simulink model "s_c107m32k_vlbi"  (R2018a)
settings: Solver=VariableStepDiscrete  StartTime=0.0  StopTime=(2^15)*10  RelTol=1e-3
undefined symbols (not defined in the file): fft_stages, n_bits_xengs
libraries: xbsIndex_r4 x23049, casper_library_misc x45, xps_library x4, casper_library_scopes x3, simulink x2
(part 45 of 201)

== system s_c107m32k_vlbi/calc_ddc_pwr1/negedge ==
  In : Inport
  Convert : xbsIndex_r4/Convert  gui_display_data_type=Fixed-point  arith_type=Boolean  n_bits=8  bin_pt=6  float_type=Single  exp_bits=8  fraction_bits=24  quantization=Truncate  overflow=Wrap  en=off  latency=0  pipeline=off  dbl_ovrd=off  block_type=convert
      settings: xl_area=[0, 0, 0, 0, 0, 0, 0]  block_version=10.1.3
  Delay : xbsIndex_r4/Delay  rst=off  infoeditControl=Selection of Reset will increase slice count due to use of real FFs and instead of SRLs  en=off  latency=1  reg_retiming=off  dbl_ovrd=off  block_type=delay
      settings: xl_area=[0, 0, 0, 0, 0, 0, 0]
  Inverter1 : xbsIndex_r4/Inverter  en=off  latency=0  dbl_ovrd=off  block_type=inv
      settings: xl_area=[0, 0, 0, 0, 0, 0, 0]
  Logical : xbsIndex_r4/Logical  logical_function=AND  inputs=2  en=off  latency=0  precision=Full  arith_type=Unsigned  n_bits=8  bin_pt=2  align_bp=on  dbl_ovrd=off  block_type=logical
      settings: xl_area=[0, 0, 0, 0, 0, 0, 0]
  Out1 : Outport
  wires:
  Inverter1/1 -> Logical/2
  Logical/1 -> Convert/1
  In/1 -> Inverter1/1, Delay/1
  Delay/1 -> Logical/1
  Convert/1 -> Out1/1

== system s_c107m32k_vlbi/calc_fft_pwr0/negedge ==
  In : Inport
  Convert : xbsIndex_r4/Convert  gui_display_data_type=Fixed-point  arith_type=Boolean  n_bits=8  bin_pt=6  float_type=Single  exp_bits=8  fraction_bits=24  quantization=Truncate  overflow=Wrap  en=off  latency=0  pipeline=off  dbl_ovrd=off  block_type=convert
      settings: xl_area=[0, 0, 0, 0, 0, 0, 0]  block_version=10.1.3
  Delay : xbsIndex_r4/Delay  rst=off  infoeditControl=Selection of Reset will increase slice count due to use of real FFs and instead of SRLs  en=off  latency=1  reg_retiming=off  dbl_ovrd=off  block_type=delay
      settings: xl_area=[0, 0, 0, 0, 0, 0, 0]
  Inverter1 : xbsIndex_r4/Inverter  en=off  latency=0  dbl_ovrd=off  block_type=inv
      settings: xl_area=[0, 0, 0, 0, 0, 0, 0]
  Logical : xbsIndex_r4/Logical  logical_function=AND  inputs=2  en=off  latency=0  precision=Full  arith_type=Unsigned  n_bits=8  bin_pt=2  align_bp=on  dbl_ovrd=off  block_type=logical
      settings: xl_area=[0, 0, 0, 0, 0, 0, 0]
  Out1 : Outport
  wires:
  Inverter1/1 -> Logical/2
  Logical/1 -> Convert/1
  In/1 -> Inverter1/1, Delay/1
  Delay/1 -> Logical/1
  Convert/1 -> Out1/1

== system s_c107m32k_vlbi/calc_fft_pwr1/negedge ==
  In : Inport
  Convert : xbsIndex_r4/Convert  gui_display_data_type=Fixed-point  arith_type=Boolean  n_bits=8  bin_pt=6  float_type=Single  exp_bits=8  fraction_bits=24  quantization=Truncate  overflow=Wrap  en=off  latency=0  pipeline=off  dbl_ovrd=off  block_type=convert
      settings: xl_area=[0, 0, 0, 0, 0, 0, 0]  block_version=10.1.3
  Delay : xbsIndex_r4/Delay  rst=off  infoeditControl=Selection of Reset will increase slice count due to use of real FFs and instead of SRLs  en=off  latency=1  reg_retiming=off  dbl_ovrd=off  block_type=delay
      settings: xl_area=[0, 0, 0, 0, 0, 0, 0]
  Inverter1 : xbsIndex_r4/Inverter  en=off  latency=0  dbl_ovrd=off  block_type=inv
      settings: xl_area=[0, 0, 0, 0, 0, 0, 0]
  Logical : xbsIndex_r4/Logical  logical_function=AND  inputs=2  en=off  latency=0  precision=Full  arith_type=Unsigned  n_bits=8  bin_pt=2  align_bp=on  dbl_ovrd=off  block_type=logical
      settings: xl_area=[0, 0, 0, 0, 0, 0, 0]
  Out1 : Outport
  wires:
  Convert/1 -> Out1/1
  Delay/1 -> Logical/1
  In/1 -> Delay/1, Inverter1/1
  Logical/1 -> Convert/1
  Inverter1/1 -> Logical/2

== system s_c107m32k_vlbi/calc_quant_pwr0/negedge ==
  In : Inport
  Convert : xbsIndex_r4/Convert  gui_display_data_type=Fixed-point  arith_type=Boolean  n_bits=8  bin_pt=6  float_type=Single  exp_bits=8  fraction_bits=24  quantization=Truncate  overflow=Wrap  en=off  latency=0  pipeline=off  dbl_ovrd=off  block_type=convert
      settings: xl_area=[0, 0, 0, 0, 0, 0, 0]  block_version=10.1.3
  Delay : xbsIndex_r4/Delay  rst=off  infoeditControl=Selection of Reset will increase slice count due to use of real FFs and instead of SRLs  en=off  latency=1  reg_retiming=off  dbl_ovrd=off  block_type=delay
      settings: xl_area=[0, 0, 0, 0, 0, 0, 0]
  Inverter1 : xbsIndex_r4/Inverter  en=off  latency=0  dbl_ovrd=off  block_type=inv
      settings: xl_area=[0, 0, 0, 0, 0, 0, 0]
  Logical : xbsIndex_r4/Logical  logical_function=AND  inputs=2  en=off  latency=0  precision=Full  arith_type=Unsigned  n_bits=8  bin_pt=2  align_bp=on  dbl_ovrd=off  block_type=logical
      settings: xl_area=[0, 0, 0, 0, 0, 0, 0]
  Out1 : Outport
  wires:
  Inverter1/1 -> Logical/2
  Logical/1 -> Convert/1
  In/1 -> Inverter1/1, Delay/1
  Delay/1 -> Logical/1
  Convert/1 -> Out1/1

== system s_c107m32k_vlbi/calc_quant_pwr1/negedge ==
  In : Inport
  Convert : xbsIndex_r4/Convert  gui_display_data_type=Fixed-point  arith_type=Boolean  n_bits=8  bin_pt=6  float_type=Single  exp_bits=8  fraction_bits=24  quantization=Truncate  overflow=Wrap  en=off  latency=0  pipeline=off  dbl_ovrd=off  block_type=convert
      settings: xl_area=[0, 0, 0, 0, 0, 0, 0]  block_version=10.1.3
  Delay : xbsIndex_r4/Delay  rst=off  infoeditControl=Selection of Reset will increase slice count due to use of real FFs and instead of SRLs  en=off  latency=1  reg_retiming=off  dbl_ovrd=off  block_type=delay
      settings: xl_area=[0, 0, 0, 0, 0, 0, 0]
  Inverter1 : xbsIndex_r4/Inverter  en=off  latency=0  dbl_ovrd=off  block_type=inv
      settings: xl_area=[0, 0, 0, 0, 0, 0, 0]
  Logical : xbsIndex_r4/Logical  logical_function=AND  inputs=2  en=off  latency=0  precision=Full  arith_type=Unsigned  n_bits=8  bin_pt=2  align_bp=on  dbl_ovrd=off  block_type=logical
      settings: xl_area=[0, 0, 0, 0, 0, 0, 0]
  Out1 : Outport
  wires:
  Convert/1 -> Out1/1
  Delay/1 -> Logical/1
  In/1 -> Delay/1, Inverter1/1
  Logical/1 -> Convert/1
  Inverter1/1 -> Logical/2

== system s_c107m32k_vlbi/cd_hmc/bus_expand1 ==
  bus_in : Inport
  reinterpret1 : xbsIndex_r4/Reinterpret  force_arith_type=on  arith_type="Signed  (2's comp)"  force_bin_pt=on  bin_pt=31  block_type=reinterpret
  reinterpret2 : xbsIndex_r4/Reinterpret  force_arith_type=on  arith_type="Signed  (2's comp)"  force_bin_pt=on  bin_pt=31  block_type=reinterpret
  reinterpret3 : xbsIndex_r4/Reinterpret  force_arith_type=on  arith_type="Signed  (2's comp)"  force_bin_pt=on  bin_pt=31  block_type=reinterpret
  reinterpret4 : xbsIndex_r4/Reinterpret  force_arith_type=on  arith_type=Unsigned  force_bin_pt=on  bin_pt=32  block_type=reinterpret
  slice1 : xbsIndex_r4/Slice  nbits=32  boolean_output=off  mode=Upper Bit Location + Width  bit1=-128  base1=MSB of Input  bit0=0  base0=LSB of Input  dbl_ovrd=off  block_type=slice
  slice2 : xbsIndex_r4/Slice  nbits=32  boolean_output=off  mode=Upper Bit Location + Width  bit1=-96  base1=MSB of Input  bit0=0  base0=LSB of Input  dbl_ovrd=off  block_type=slice
  slice3 : xbsIndex_r4/Slice  nbits=32  boolean_output=off  mode=Upper Bit Location + Width  bit1=-64  base1=MSB of Input  bit0=0  base0=LSB of Input  dbl_ovrd=off  block_type=slice
  slice4 : xbsIndex_r4/Slice  nbits=64  boolean_output=off  mode=Upper Bit Location + Width  bit1=0  base1=MSB of Input  bit0=0  base0=LSB of Input  dbl_ovrd=off  block_type=slice
  msb_out4 : Outport
  out3 : Outport  Port=2
  out2 : Outport  Port=3
  lsb_out1 : Outport  Port=4
  wires:
  reinterpret1/1 -> lsb_out1/1
  slice1/1 -> reinterpret1/1
  reinterpret2/1 -> out2/1
  slice2/1 -> reinterpret2/1
  reinterpret3/1 -> out3/1
  slice3/1 -> reinterpret3/1
  reinterpret4/1 -> msb_out4/1
  slice4/1 -> reinterpret4/1
  bus_in/1 -> slice1/1, slice2/1, slice3/1, slice4/1

== system s_c107m32k_vlbi/cd_hmc/bus_expand2 ==
  bus_in : Inport
  reinterpret1 : xbsIndex_r4/Reinterpret  force_arith_type=on  arith_type="Signed  (2's comp)"  force_bin_pt=on  bin_pt=31  block_type=reinterpret
  reinterpret2 : xbsIndex_r4/Reinterpret  force_arith_type=on  arith_type="Signed  (2's comp)"  force_bin_pt=on  bin_pt=31  block_type=reinterpret
  reinterpret3 : xbsIndex_r4/Reinterpret  force_arith_type=on  arith_type="Signed  (2's comp)"  force_bin_pt=on  bin_pt=31  block_type=reinterpret
  reinterpret4 : xbsIndex_r4/Reinterpret  force_arith_type=on  arith_type=Unsigned  force_bin_pt=on  bin_pt=32  block_type=reinterpret
  slice1 : xbsIndex_r4/Slice  nbits=32  boolean_output=off  mode=Upper Bit Location + Width  bit1=-128  base1=MSB of Input  bit0=0  base0=LSB of Input  dbl_ovrd=off  block_type=slice
  slice2 : xbsIndex_r4/Slice  nbits=32  boolean_output=off  mode=Upper Bit Location + Width  bit1=-96  base1=MSB of Input  bit0=0  base0=LSB of Input  dbl_ovrd=off  block_type=slice
  slice3 : xbsIndex_r4/Slice  nbits=32  boolean_output=off  mode=Upper Bit Location + Width  bit1=-64  base1=MSB of Input  bit0=0  base0=LSB of Input  dbl_ovrd=off  block_type=slice
  slice4 : xbsIndex_r4/Slice  nbits=64  boolean_output=off  mode=Upper Bit Location + Width  bit1=0  base1=MSB of Input  bit0=0  base0=LSB of Input  dbl_ovrd=off  block_type=slice
  msb_out4 : Outport
  out3 : Outport  Port=2
  out2 : Outport  Port=3
  lsb_out1 : Outport  Port=4
  wires:
  reinterpret1/1 -> lsb_out1/1
  slice1/1 -> reinterpret1/1
  reinterpret2/1 -> out2/1
  slice2/1 -> reinterpret2/1
  reinterpret3/1 -> out3/1
  slice3/1 -> reinterpret3/1
  reinterpret4/1 -> msb_out4/1
  slice4/1 -> reinterpret4/1
  bus_in/1 -> slice1/1, slice2/1, slice3/1, slice4/1

== system s_c107m32k_vlbi/cd_hmc/delay_gen0 ==
  note: Make space here (cast) for the upcoming
      | scaling, ensuring that we keep the
      | required precision.
      | Shift phase and delay rates down
      | to fit into specified range.
      | An update is only done at the end of
      | every FFT spectrum so modify shift to
      | not be as large
  note: Need negative slope
      | for positive deay
  note: Extract whole part
  note: Extract fractional part
  note: coarse delay rotates phase around 0th
      | channel. We want to reference with respect to
      | centre of band. So subtract half the coarse
      | delay amount.
  sync_in : Inport
  init : Inport  Port=2
  din : Inport  Port=3
  idx_in : Inport  Port=4
  den : Inport  Port=5
  load : Inport  Port=6
  phase : Inport  Port=7
  d/dt_phase : Inport  Port=8
  delay : Inport  Port=9
  d/dt_delay : Inport  Port=10
  invert_slope : Inport  Port=11
  AddSub : xbsIndex_r4/AddSub  mode=Addition  use_carryin=off  use_carryout=off  en=off  latency=1  precision=Full  arith_type=Unsigned  n_bits=16  bin_pt=14  quantization=Truncate  overflow=Wrap  use_behavioral_HDL=on  hw_selection=Fabric  pipelined=off  dbl_ovrd=off  block_type=addsub
  Concat : xbsIndex_r4/Concat  num_inputs=4  dbl_ovrd=off  block_type=concat
  Constant : xbsIndex_r4/Constant  const=1  gui_display_data_type=Fixed-point  arith_type=Unsigned  n_bits=1  bin_pt=0  preci_type=Single  exp_width=8  frac_width=24  explicit_period=on  period=1  equ=P=C  opselect=C  inp2=PCIN>>17  opr=+  inp1=P  carry=CIN  dbl_ovrd=off  block_type=constant
  Convert : xbsIndex_r4/Convert  gui_display_data_type=Fixed-point  arith_type="Signed  (2's comp)"  n_bits=comp_phase_rate_bits  bin_pt=comp_phase_rate_bin_pt  float_type=Single  exp_bits=8  fraction_bits=24  quantization="Round  (unbiased: +/- Inf)"  overflow=Saturate  en=off  latency=0  pipeline=off  dbl_ovrd=off  block_type=convert
  Convert1 : xbsIndex_r4/Convert  gui_display_data_type=Fixed-point  arith_type="Signed  (2's comp)"  n_bits=comp_delay_rate_bits  bin_pt=comp_delay_rate_bin_pt  float_type=Single  exp_bits=8  fraction_bits=24  quantization="Round  (unbiased: +/- Inf)"  overflow=Saturate  en=off  latency=0  pipeline=off  dbl_ovrd=off  block_type=convert
  Convert4 : xbsIndex_r4/Convert  gui_display_data_type=Fixed-point  arith_type="Signed  (2's comp)"  n_bits=max(phase_bits, comp_phase_rate_bits)  bin_pt=max(phase_bits-1, comp_phase_rate_bin_pt)  float_type=Single  exp_bits=8  fraction_bits=24  quantization=Truncate  overflow=Wrap  en=off  latency=1  pipeline=on  dbl_ovrd=off  block_type=convert
      settings: block_version=10.1.3
  Convert5 : xbsIndex_r4/Convert  gui_display_data_type=Fixed-point  arith_type=Unsigned  n_bits=cd_bits  bin_pt=0  float_type=Single  exp_bits=8  fraction_bits=24  quantization=Truncate  overflow=Wrap  en=off  latency=1  pipeline=on  dbl_ovrd=off  block_type=convert
      settings: block_version=10.1.3
  Convert6 : xbsIndex_r4/Convert  gui_display_data_type=Fixed-point  arith_type=Unsigned  n_bits=max(delay_bin_pt, comp_delay_rate_bin_pt)  bin_pt=max(delay_bin_pt, comp_delay_rate_bin_pt)  float_type=Single  exp_bits=8  fraction_bits=24  quantization=Truncate  overflow=Wrap  en=off  latency=1  pipeline=on  dbl_ovrd=off  block_type=convert
      settings: block_version=10.1.3
  Delay{1..14,16} (15 alike) : xbsIndex_r4/Delay  rst=off  infoeditControl=Selection of Reset will increase slice count due to use of real FFs and instead of SRLs  en=off  latency=1  reg_retiming=on  dbl_ovrd=off  block_type=delay
      settings: block_version=11.4
  Mux : xbsIndex_r4/Mux  inputs=2  en=off  latency=1  precision=Full  arith_type=Unsigned  n_bits=16  bin_pt=14  quantization=Truncate  overflow=Wrap  dbl_ovrd=off  block_type=mux
      settings: block_version=11.4
  Negate : xbsIndex_r4/Negate  precision=Full  arith_type="Signed  (2's comp)"  n_bits=lookup_bits + fft_len  bin_pt=lookup_bits + fft_len - 1  quantization=Truncate  overflow=Saturate  en=off  latency=1  dbl_ovrd=off  block_type=negate
      settings: block_version=11.4
  Reinterpret{,1..3} (4 alike) : xbsIndex_r4/Reinterpret  force_arith_type=on  arith_type=Unsigned  force_bin_pt=on  bin_pt=0  block_type=reinterpret
  Slice5 : xbsIndex_r4/Slice  nbits=2  boolean_output=off  mode=Lower Bit Location + Width  bit1=0  base1=MSB of Input  bit0=0  base0=LSB of Input  dbl_ovrd=off  block_type=slice
  Terminator : Terminator
  Terminator1 : Terminator
  bus_expand : Subsystem  AncestorBlock=casper_library_flow_control/bus_expand  mask(bus_expand){mode=divisions of arbitrary size, outputNum=1, outputWidth=[1 1 data_bits n_bits_index], outputBinaryPt=[0 0 0 0], outputArithmeticType=[2 2 0 0], show_format=off, outputToWorkspace=off, variablePrefix=out, outputToModelAsWell=on}
      mask prompts: outputNum "Number of outputs:"; outputWidth "Output width [msb ... lsb]:"; outputBinaryPt "Output binary point position [msb ... lsb]:"; outputArithmeticType "Output arithmetic type (ufix=0, fix=1, bool=2) [msb ... lsb]:"; show_format "Print format string?"; outputToWorkspace "Output to workspace?"; variablePrefix "Variable name prefix:"; outputToModelAsWell "Output to model as well?"
      mask help:
      | Expands a 'bus' made using a bus_create or Xilinx
      | concat block.
      | The input will be divided into the specified number
      | of outputs with the specified arithmetic types.
      | Divisions are made from most significant bit.
      mask init: same as s_c107m32k_vlbi/bus_expand1
      settings: AttributesFormatString=4 outputs
      mask TypeOptions mode: divisions of equal size | divisions of arbitrary size
      mask Callback mode: bus_expand_callback();
      mask Callback outputWidth: bus_expand_callback();
      mask Callback outputToWorkspace: bus_expand_callback();
  delay_calc : Subsystem  mask{bit_width=max(delay_bits, comp_delay_rate_bits), bin_pt=max(delay_bin_pt, comp_delay_rate_bin_pt)}
      mask prompts: bit_width "Coefficient bit width"; bin_pt "Coefficient binary point"
  half_cd : xbsIndex_r4/Shift  shift_dir=Right  shift_bits=1  en=off  latency=0  precision=User Defined  arith_type=Unsigned  n_bits=2  bin_pt=1  quantization=Truncate  overflow=Saturate  dbl_ovrd=off  block_type=shift
  normalise+fft0 : xbsIndex_r4/Shift  shift_dir=Right  shift_bits=phase_rate_scale_factor  en=off  latency=0  precision=Full  arith_type="Signed  (2's comp)"  n_bits=comp_phase_rate_bits  bin_pt=comp_phase_rate_bin_pt  quantization="Round  (unbiased: +/- Inf)"  overflow=Saturate  dbl_ovrd=off  block_type=shift
  normalise+fft1 : xbsIndex_r4/Shift  shift_dir=Right  shift_bits=delay_rate_scale_factor  en=off  latency=0  precision=Full  arith_type="Signed  (2's comp)"  n_bits=comp_delay_rate_bits  bin_pt=comp_delay_rate_bin_pt  quantization="Round  (unbiased: +/- Inf)"  overflow=Saturate  dbl_ovrd=off  block_type=shift
  phase_calc : Subsystem  mask{bit_width=max(phase_bits, comp_phase_rate_bits), bin_pt=max(phase_bits-1, comp_phase_rate_bin_pt)}
      mask prompts: bit_width "Coefficient bit width"; bin_pt "Coefficient binary point"
  sync_out : Outport
  dout : Outport  Port=2
  idx_out : Outport  Port=3
  dvalid : Outport  Port=4
  cd_o : Outport  Port=5
  slope_out : Outport  Port=6
  phase_out : Outport  Port=7
  load_out : Outport  Port=8
  wires:
  d/dt_delay/1 -> Convert1/1
  normalise+fft1/1 -> delay_calc/3(val_inc)
  d/dt_phase/1 -> Convert/1
  Delay16/1 -> Delay14/1
  Delay2/1 -> Delay7/1
  Convert4/1 -> Delay10/1
  Mux/1 -> slope_out/1
  Convert6/1 -> Delay13/1, Negate/1
  delay_calc/3(en_o) -> Terminator/1
  phase_calc/3(en_o) -> Delay1/1
  delay_calc/2(coeff) -> Delay12/1, Convert5/1
  [tick] -> delay_calc/5(update)
  [tick] -> phase_calc/5(update)
  [en] -> delay_calc/4(en)
  [en] -> phase_calc/4(en)
  normalise+fft0/1 -> phase_calc/3(val_inc)
  load/1 -> [en]
  Delay4/1 -> Delay2/1
  Delay5/1 -> Delay16/1
  invert_slope/1 -> Mux/1
  Negate/1 -> Mux/2
  Delay8/1 -> Delay9/1
  init/1 -> [tick]
  sync_in/1 -> Reinterpret/1
  Concat/1 -> phase_calc/1(din)
  Convert5/1 -> Slice5/1, Delay5/1
  Slice5/1 -> half_cd/1
  half_cd/1 -> AddSub/2
  phase_calc/2(coeff) -> Delay3/1
  AddSub/1 -> Convert4/1
  phase_calc/1(dout) -> Delay11/1
  Delay9/1 -> Delay6/1
  Delay1/1 -> Delay4/1
  Delay3/1 -> AddSub/1
  Delay11/1 -> Delay8/1
  Delay12/1 -> Convert6/1
  phase/1 -> phase_calc/2(val)
  delay/1 -> delay_calc/2(val)
  Constant/1 -> delay_calc/1(din)
  delay_calc/1(dout) -> Terminator1/1
  Delay13/1 -> Mux/3
  Reinterpret/1 -> Concat/1
  Reinterpret1/1 -> Concat/2
  Reinterpret2/1 -> Concat/3
  Reinterpret3/1 -> Concat/4
  bus_expand/1(msb_out4) -> sync_out/1
  den/1 -> Reinterpret1/1
  din/1 -> Reinterpret2/1
  idx_in/1 -> Reinterpret3/1
  bus_expand/2(out3) -> dvalid/1
  bus_expand/3(out2) -> dout/1
  bus_expand/4(lsb_out1) -> idx_out/1
  Delay6/1 -> bus_expand/1(bus_in)
  Delay7/1 -> load_out/1
  Delay10/1 -> phase_out/1
  Delay14/1 -> cd_o/1
  Convert/1 -> normalise+fft0/1
  Convert1/1 -> normalise+fft1/1

== system s_c107m32k_vlbi/cd_hmc/delay_gen1 ==
  note: coarse delay rotates phase around 0th
      | channel. We want to reference with respect to
      | centre of band. So subtract half the coarse
      | delay amount.
  note: Extract fractional part
  note: Extract whole part
  note: Need negative slope
      | for positive deay
  note: Make space here (cast) for the upcoming
      | scaling, ensuring that we keep the
      | required precision.
      | Shift phase and delay rates down
      | to fit into specified range.
      | An update is only done at the end of
      | every FFT spectrum so modify shift to
      | not be as large
  sync_in : Inport
  init : Inport  Port=2
  din : Inport  Port=3
  idx_in : Inport  Port=4
  den : Inport  Port=5
  load : Inport  Port=6
  phase : Inport  Port=7
  d/dt_phase : Inport  Port=8
  delay : Inport  Port=9
  d/dt_delay : Inport  Port=10
  invert_slope : Inport  Port=11
  AddSub : xbsIndex_r4/AddSub  mode=Addition  use_carryin=off  use_carryout=off  en=off  latency=1  precision=Full  arith_type=Unsigned  n_bits=16  bin_pt=14  quantization=Truncate  overflow=Wrap  use_behavioral_HDL=on  hw_selection=Fabric  pipelined=off  dbl_ovrd=off  block_type=addsub
  Concat : xbsIndex_r4/Concat  num_inputs=4  dbl_ovrd=off  block_type=concat
  Constant : xbsIndex_r4/Constant  const=1  gui_display_data_type=Fixed-point  arith_type=Unsigned  n_bits=1  bin_pt=0  preci_type=Single  exp_width=8  frac_width=24  explicit_period=on  period=1  equ=P=C  opselect=C  inp2=PCIN>>17  opr=+  inp1=P  carry=CIN  dbl_ovrd=off  block_type=constant
  Convert : xbsIndex_r4/Convert  gui_display_data_type=Fixed-point  arith_type="Signed  (2's comp)"  n_bits=comp_phase_rate_bits  bin_pt=comp_phase_rate_bin_pt  float_type=Single  exp_bits=8  fraction_bits=24  quantization="Round  (unbiased: +/- Inf)"  overflow=Saturate  en=off  latency=0  pipeline=off  dbl_ovrd=off  block_type=convert
  Convert1 : xbsIndex_r4/Convert  gui_display_data_type=Fixed-point  arith_type="Signed  (2's comp)"  n_bits=comp_delay_rate_bits  bin_pt=comp_delay_rate_bin_pt  float_type=Single  exp_bits=8  fraction_bits=24  quantization="Round  (unbiased: +/- Inf)"  overflow=Saturate  en=off  latency=0  pipeline=off  dbl_ovrd=off  block_type=convert
  Convert4 : xbsIndex_r4/Convert  gui_display_data_type=Fixed-point  arith_type="Signed  (2's comp)"  n_bits=max(phase_bits, comp_phase_rate_bits)  bin_pt=max(phase_bits-1, comp_phase_rate_bin_pt)  float_type=Single  exp_bits=8  fraction_bits=24  quantization=Truncate  overflow=Wrap  en=off  latency=1  pipeline=on  dbl_ovrd=off  block_type=convert
      settings: block_version=10.1.3
  Convert5 : xbsIndex_r4/Convert  gui_display_data_type=Fixed-point  arith_type=Unsigned  n_bits=cd_bits  bin_pt=0  float_type=Single  exp_bits=8  fraction_bits=24  quantization=Truncate  overflow=Wrap  en=off  latency=1  pipeline=on  dbl_ovrd=off  block_type=convert
      settings: block_version=10.1.3
  Convert6 : xbsIndex_r4/Convert  gui_display_data_type=Fixed-point  arith_type=Unsigned  n_bits=max(delay_bin_pt, comp_delay_rate_bin_pt)  bin_pt=max(delay_bin_pt, comp_delay_rate_bin_pt)  float_type=Single  exp_bits=8  fraction_bits=24  quantization=Truncate  overflow=Wrap  en=off  latency=1  pipeline=on  dbl_ovrd=off  block_type=convert
      settings: block_version=10.1.3
  Delay{1..14,16} (15 alike) : xbsIndex_r4/Delay  rst=off  infoeditControl=Selection of Reset will increase slice count due to use of real FFs and instead of SRLs  en=off  latency=1  reg_retiming=on  dbl_ovrd=off  block_type=delay
      settings: block_version=11.4
  Mux : xbsIndex_r4/Mux  inputs=2  en=off  latency=1  precision=Full  arith_type=Unsigned  n_bits=16  bin_pt=14  quantization=Truncate  overflow=Wrap  dbl_ovrd=off  block_type=mux
      settings: block_version=11.4
  Negate : xbsIndex_r4/Negate  precision=Full  arith_type="Signed  (2's comp)"  n_bits=lookup_bits + fft_len  bin_pt=lookup_bits + fft_len - 1  quantization=Truncate  overflow=Saturate  en=off  latency=1  dbl_ovrd=off  block_type=negate
      settings: block_version=11.4
  Reinterpret{,1..3} (4 alike) : xbsIndex_r4/Reinterpret  force_arith_type=on  arith_type=Unsigned  force_bin_pt=on  bin_pt=0  block_type=reinterpret
  Slice5 : xbsIndex_r4/Slice  nbits=2  boolean_output=off  mode=Lower Bit Location + Width  bit1=0  base1=MSB of Input  bit0=0  base0=LSB of Input  dbl_ovrd=off  block_type=slice
  Terminator : Terminator
  Terminator1 : Terminator
  bus_expand : Subsystem  AncestorBlock=casper_library_flow_control/bus_expand  mask(bus_expand){mode=divisions of arbitrary size, outputNum=1, outputWidth=[1 1 data_bits n_bits_index], outputBinaryPt=[0 0 0 0], outputArithmeticType=[2 2 0 0], show_format=off, outputToWorkspace=off, variablePrefix=out, outputToModelAsWell=on}
      mask prompts: outputNum "Number of outputs:"; outputWidth "Output width [msb ... lsb]:"; outputBinaryPt "Output binary point position [msb ... lsb]:"; outputArithmeticType "Output arithmetic type (ufix=0, fix=1, bool=2) [msb ... lsb]:"; show_format "Print format string?"; outputToWorkspace "Output to workspace?"; variablePrefix "Variable name prefix:"; outputToModelAsWell "Output to model as well?"
      mask help:
      | Expands a 'bus' made using a bus_create or Xilinx
      | concat block.
      | The input will be divided into the specified number
      | of outputs with the specified arithmetic types.
      | Divisions are made from most significant bit.
      mask init: same as s_c107m32k_vlbi/bus_expand1
      settings: AttributesFormatString=4 outputs
      mask TypeOptions mode: divisions of equal size | divisions of arbitrary size
      mask Callback mode: bus_expand_callback();
      mask Callback outputWidth: bus_expand_callback();
      mask Callback outputToWorkspace: bus_expand_callback();
  delay_calc : Subsystem  mask{bit_width=max(delay_bits, comp_delay_rate_bits), bin_pt=max(delay_bin_pt, comp_delay_rate_bin_pt)}
      mask prompts: bit_width "Coefficient bit width"; bin_pt "Coefficient binary point"
  half_cd : xbsIndex_r4/Shift  shift_dir=Right  shift_bits=1  en=off  latency=0  precision=User Defined  arith_type=Unsigned  n_bits=2  bin_pt=1  quantization=Truncate  overflow=Saturate  dbl_ovrd=off  block_type=shift
  normalise+fft0 : xbsIndex_r4/Shift  shift_dir=Right  shift_bits=phase_rate_scale_factor  en=off  latency=0  precision=Full  arith_type="Signed  (2's comp)"  n_bits=comp_phase_rate_bits  bin_pt=comp_phase_rate_bin_pt  quantization="Round  (unbiased: +/- Inf)"  overflow=Saturate  dbl_ovrd=off  block_type=shift
  normalise+fft1 : xbsIndex_r4/Shift  shift_dir=Right  shift_bits=delay_rate_scale_factor  en=off  latency=0  precision=Full  arith_type="Signed  (2's comp)"  n_bits=comp_delay_rate_bits  bin_pt=comp_delay_rate_bin_pt  quantization="Round  (unbiased: +/- Inf)"  overflow=Saturate  dbl_ovrd=off  block_type=shift
  phase_calc : Subsystem  mask{bit_width=max(phase_bits, comp_phase_rate_bits), bin_pt=max(phase_bits-1, comp_phase_rate_bin_pt)}
      mask prompts: bit_width "Coefficient bit width"; bin_pt "Coefficient binary point"
  sync_out : Outport
  dout : Outport  Port=2
  idx_out : Outport  Port=3
  dvalid : Outport  Port=4
  cd_o : Outport  Port=5
  slope_out : Outport  Port=6
  phase_out : Outport  Port=7
  load_out : Outport  Port=8
  wires:
  Convert1/1 -> normalise+fft1/1
  Convert/1 -> normalise+fft0/1
  Delay14/1 -> cd_o/1
  Delay10/1 -> phase_out/1
  Delay7/1 -> load_out/1
  Delay6/1 -> bus_expand/1(bus_in)
  bus_expand/4(lsb_out1) -> idx_out/1
  bus_expand/3(out2) -> dout/1
  bus_expand/2(out3) -> dvalid/1
  idx_in/1 -> Reinterpret3/1
  din/1 -> Reinterpret2/1
  den/1 -> Reinterpret1/1
  bus_expand/1(msb_out4) -> sync_out/1
  Reinterpret3/1 -> Concat/4
  Reinterpret2/1 -> Concat/3
  Reinterpret1/1 -> Concat/2
  Reinterpret/1 -> Concat/1
  Delay13/1 -> Mux/3
  delay_calc/1(dout) -> Terminator1/1
  Constant/1 -> delay_calc/1(din)
  delay/1 -> delay_calc/2(val)
  phase/1 -> phase_calc/2(val)
  Delay12/1 -> Convert6/1
  Delay11/1 -> Delay8/1
  Delay3/1 -> AddSub/1
  Delay1/1 -> Delay4/1
  Delay9/1 -> Delay6/1
  phase_calc/1(dout) -> Delay11/1
  AddSub/1 -> Convert4/1
  phase_calc/2(coeff) -> Delay3/1
  half_cd/1 -> AddSub/2
  Slice5/1 -> half_cd/1
  Convert5/1 -> Delay5/1, Slice5/1
  Concat/1 -> phase_calc/1(din)
  sync_in/1 -> Reinterpret/1
  init/1 -> [tick]
  Delay8/1 -> Delay9/1
  Negate/1 -> Mux/2
  invert_slope/1 -> Mux/1
  Delay5/1 -> Delay16/1
  Delay4/1 -> Delay2/1
  load/1 -> [en]
  normalise+fft0/1 -> phase_calc/3(val_inc)
  [en] -> phase_calc/4(en)
  [en] -> delay_calc/4(en)
  [tick] -> phase_calc/5(update)
  [tick] -> delay_calc/5(update)
  delay_calc/2(coeff) -> Convert5/1, Delay12/1
  phase_calc/3(en_o) -> Delay1/1
  delay_calc/3(en_o) -> Terminator/1
  Convert6/1 -> Negate/1, Delay13/1
  Mux/1 -> slope_out/1
  Convert4/1 -> Delay10/1
  Delay2/1 -> Delay7/1
  Delay16/1 -> Delay14/1
  d/dt_phase/1 -> Convert/1
  normalise+fft1/1 -> delay_calc/3(val_inc)
  d/dt_delay/1 -> Convert1/1

== system s_c107m32k_vlbi/cd_hmc/edge_detect ==
  in : Inport
  Delay : xbsIndex_r4/Delay  rst=off  infoeditControl=Selection of Reset will increase slice count due to use of real FFs and instead of SRLs  en=off  latency=1  reg_retiming=off  dbl_ovrd=off  block_type=delay
      settings: xl_area=[0, 0, 0, 0, 0, 0, 0]
  Inverter : xbsIndex_r4/Inverter  en=off  latency=0  dbl_ovrd=off  block_type=inv
      settings: xl_area=[0, 0, 0, 0, 0, 0, 0]
  edge_op : xbsIndex_r4/Logical  logical_function=NOR  inputs=2  en=off  latency=0  precision=Full  arith_type=Unsigned  n_bits=8  bin_pt=2  align_bp=on  dbl_ovrd=off  block_type=logical
      settings: xl_area=[0, 0, 0, 0, 0, 0, 0]
  out : Outport
  wires:
  Delay/1 -> edge_op/2
  in/1 -> Delay/1, Inverter/1
  edge_op/1 -> out/1
  Inverter/1 -> edge_op/1

== system s_c107m32k_vlbi/cd_hmc/edge_detect1 ==
  in : Inport
  Delay : xbsIndex_r4/Delay  rst=off  infoeditControl=Selection of Reset will increase slice count due to use of real FFs and instead of SRLs  en=off  latency=1  reg_retiming=off  dbl_ovrd=off  block_type=delay
      settings: xl_area=[0, 0, 0, 0, 0, 0, 0]
  Inverter : xbsIndex_r4/Inverter  en=off  latency=0  dbl_ovrd=off  block_type=inv
      settings: xl_area=[0, 0, 0, 0, 0, 0, 0]
  edge_op : xbsIndex_r4/Logical  logical_function=NOR  inputs=2  en=off  latency=0  precision=Full  arith_type=Unsigned  n_bits=8  bin_pt=2  align_bp=on  dbl_ovrd=off  block_type=logical
      settings: xl_area=[0, 0, 0, 0, 0, 0, 0]
  out : Outport
  wires:
  Delay/1 -> edge_op/2
  in/1 -> Delay/1, Inverter/1
  edge_op/1 -> out/1
  Inverter/1 -> edge_op/1

== system s_c107m32k_vlbi/cd_hmc/edge_detect2 ==
  in : Inport
  Delay : xbsIndex_r4/Delay  rst=off  infoeditControl=Selection of Reset will increase slice count due to use of real FFs and instead of SRLs  en=off  latency=1  reg_retiming=off  dbl_ovrd=off  block_type=delay
      settings: xl_area=[0, 0, 0, 0, 0, 0, 0]
  Inverter : xbsIndex_r4/Inverter  en=off  latency=0  dbl_ovrd=off  block_type=inv
      settings: xl_area=[0, 0, 0, 0, 0, 0, 0]
  edge_op : xbsIndex_r4/Logical  logical_function=NOR  inputs=2  en=off  latency=0  precision=Full  arith_type=Unsigned  n_bits=8  bin_pt=2  align_bp=on  dbl_ovrd=off  block_type=logical
      settings: xl_area=[0, 0, 0, 0, 0, 0, 0]
  out : Outport
  wires:
  Inverter/1 -> edge_op/1
  edge_op/1 -> out/1
  in/1 -> Inverter/1, Delay/1
  Delay/1 -> edge_op/2
